simulink model "rl"  (R2020b)
settings: Solver=FixedStepAuto  StartTime=0.0  StopTime=100  FixedStep=0.1  RelTol=1e-3
libraries: rllib x1, simulink_extras x1
settings Model: Creator=Kazemi  LastModifiedBy=Kazemi

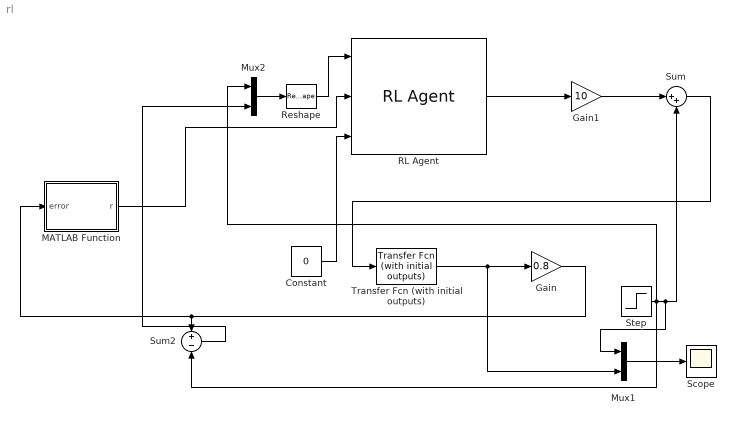
== system rl ==
  Constant : Constant  Value=0
  Gain : Gain  Gain=0.8
  Gain1 : Gain  Gain=10
  MATLAB Function : MATLAB Function  TreatAsAtomicUnit=on
  Mux1 : Mux  Inputs=3
  Mux2 : Mux  Inputs=2
  RL Agent : rllib/RL Agent  Agent=agentObj  ProvideReward=on  ProvideIsDone=on  ProvideCumRwd=off  TreatAsDirectFeedthrough=on  CollectLoggedSignals=on  CollectModelStates=on
  Reshape : Reshape  OutputDimensionality=Column vector (2-D)
  Scope : Scope
  Step : Step  Time=10  After=10  SampleTime=0
  Sum : Sum  Inputs=|++
  Sum2 : Sum  Inputs=+-
  Transfer Fcn (with initial outputs) : simulink_extras/Additional Linear/Transfer Fcn (with initial outputs)  N=[1]  D=[0.5 1]  Y0=.5  U0=0
  wires:
  RL Agent/1 -> Gain1/1
  Gain1/1 -> Sum/1
  Step/1 -> Sum2/2, Mux2/1, Mux1/1, Sum/2
  Transfer Fcn (with initial outputs)/1 -> Mux1/3, Gain/1
  Sum/1 -> Transfer Fcn (with initial outputs)/1
  Gain/1 -> MATLAB Function/1(error), Sum2/1
  Sum2/1 -> Mux2/2
  Constant/1 -> RL Agent/3
  Mux1/1 -> Scope/1
  Reshape/1 -> RL Agent/1
  Mux2/1 -> Reshape/1
  MATLAB Function/1(r) -> RL Agent/2

== matlab function rl/MATLAB Function ==
  data: error input; r output
function r = fcn(error)
    % فرمول مقاله: ترکیبی از توان ۲ و تانژانت هیپربولیک
    % هدف: مجازات کردن خطا (هرچه خطا بیشتر، عدد منفی‌تر)
    
    e_sq = error^2;
    r = -100 * (0.05 * e_sq + 0.45 * tanh(e_sq));
    
    % نکته: من یک ضریب ۱۰۰ اضافه کردم تا پاداش‌ها بزرگتر بشن 
    % و ایجنت سریع‌تر بفهمه مسیر درست کدومه.
end
